simulink model "hw2_model"  (R2024b)
settings: Solver=FixedStepAuto  StartTime=0.0  StopTime=T  FixedStep=dt  RelTol=1e-3
undefined symbols (not defined in the file): dt, L, P0, Q, R, x0
settings Model: Creator=Atakan  LastModifiedBy=Atakan

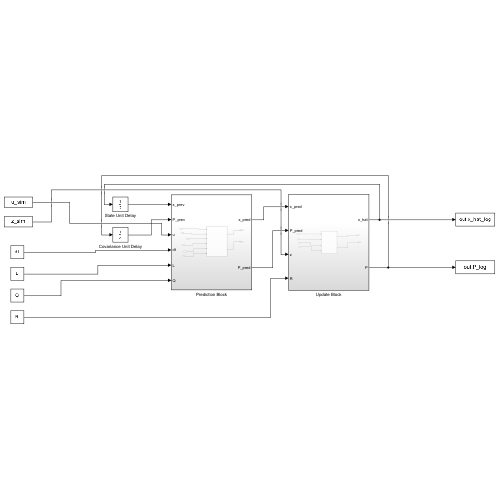
[thumbnail: Simulink's stored preview of the top-level diagram]
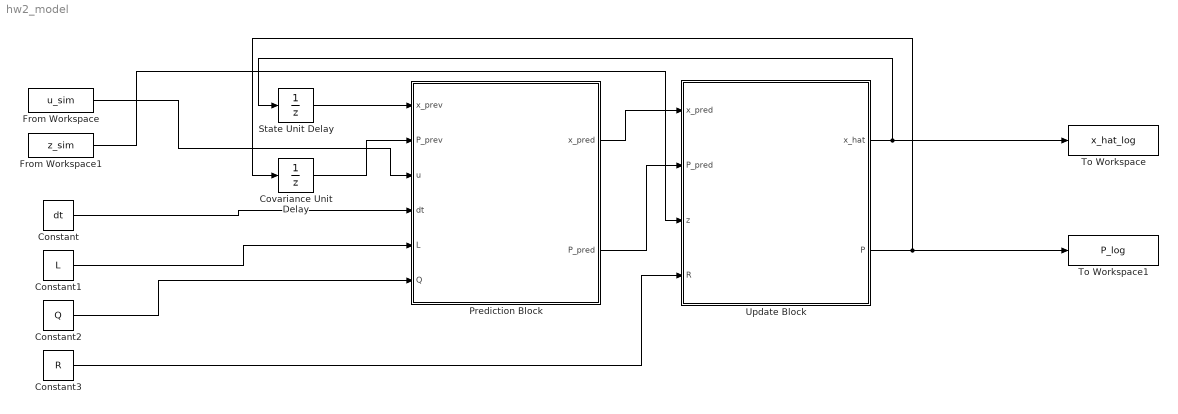
== system hw2_model ==
  Constant : Constant  Value=dt
  Constant1 : Constant  Value=L
  Constant2 : Constant  Value=Q
  Constant3 : Constant  Value=R
  Covariance Unit Delay : UnitDelay  InitialCondition=P0  SampleTime=dt  HasFrameUpgradeWarning=on
  From Workspace : FromWorkspace  VariableName=u_sim
  From Workspace1 : FromWorkspace  VariableName=z_sim
  Prediction Block : Subsystem
  State Unit Delay : UnitDelay  InitialCondition=x0  SampleTime=dt  HasFrameUpgradeWarning=on
  To Workspace : ToWorkspace  VariableName=x_hat_log  SampleTime=-1
  To Workspace1 : ToWorkspace  VariableName=P_log  SampleTime=-1
  Update Block : Subsystem
  wires:
  State Unit Delay/1 -> Prediction Block/1(x_prev)
  Covariance Unit Delay/1 -> Prediction Block/2(P_prev)
  From Workspace/1 -> Prediction Block/3(u)
  Constant/1 -> Prediction Block/4(dt)
  Constant1/1 -> Prediction Block/5(L)
  Constant2/1 -> Prediction Block/6(Q)
  Prediction Block/1(x_pred) -> Update Block/1(x_pred)
  Prediction Block/2(P_pred) -> Update Block/2(P_pred)
  From Workspace1/1 -> Update Block/3(z)
  Constant3/1 -> Update Block/4(R)
  Update Block/1(x_hat) -> State Unit Delay/1, To Workspace/1
  Update Block/2(P) -> To Workspace1/1, Covariance Unit Delay/1

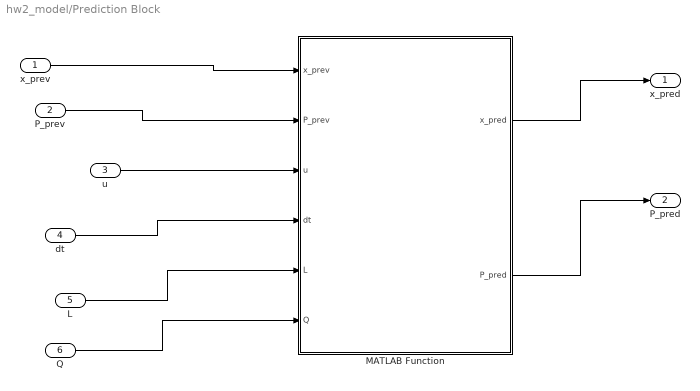
== system hw2_model/Prediction Block ==
  x_prev : Inport
  P_prev : Inport  Port=2
  u : Inport  Port=3
  dt : Inport  Port=4
  L : Inport  Port=5
  Q : Inport  Port=6
  MATLAB Function : MATLAB Function  TreatAsAtomicUnit=on
  x_pred : Outport
  P_pred : Outport  Port=2
  wires:
  x_prev/1 -> MATLAB Function/1(x_prev)
  P_prev/1 -> MATLAB Function/2(P_prev)
  u/1 -> MATLAB Function/3(u)
  dt/1 -> MATLAB Function/4(dt)
  L/1 -> MATLAB Function/5(L)
  Q/1 -> MATLAB Function/6(Q)
  MATLAB Function/1(x_pred) -> x_pred/1
  MATLAB Function/2(P_pred) -> P_pred/1

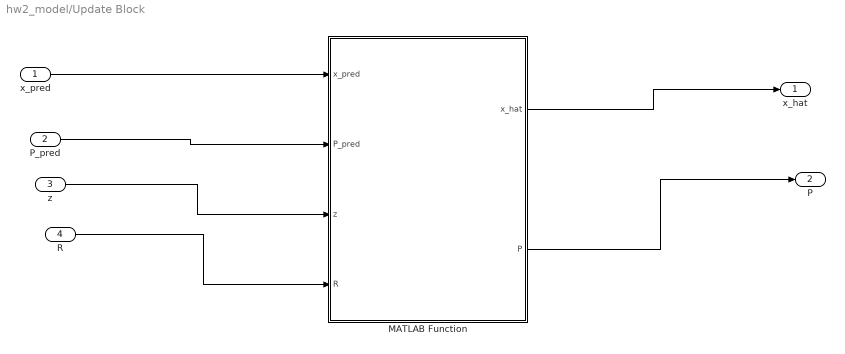
== system hw2_model/Update Block ==
  x_pred : Inport
  P_pred : Inport  Port=2
  z : Inport  Port=3
  R : Inport  Port=4
  MATLAB Function : MATLAB Function  TreatAsAtomicUnit=on
  x_hat : Outport
  P : Outport  Port=2
  wires:
  x_pred/1 -> MATLAB Function/1(x_pred)
  P_pred/1 -> MATLAB Function/2(P_pred)
  z/1 -> MATLAB Function/3(z)
  R/1 -> MATLAB Function/4(R)
  MATLAB Function/1(x_hat) -> x_hat/1
  MATLAB Function/2(P) -> P/1

== matlab function hw2_model/Update Block/MATLAB Function ==
  data: x_pred input; x_hat output; P_pred input; z input; R input; P output
function [x_hat, P] = update_block(x_pred, P_pred, z, R)
% EKF update step for GPS-like position measurement

% Make measurement vector safe
z = z(:);

% Measurement matrix
H = [1, 0, 0;
     0, 1, 0];

% Predicted measurement
z_pred = H*x_pred;

% Innovation
y = z - z_pred;

% Innovation covariance
S = H*P_pred*H' + R;

% Kalman gain
K = (P_pred*H') / S;

% State update
x_hat = x_pred + K*y;

% Normalize heading angle
x_hat(3) = atan2(sin(x_hat(3)), cos(x_hat(3)));

% Covariance update
I = eye(3);
P = (I - K*H)*P_pred;
end

== matlab function hw2_model/Prediction Block/MATLAB Function ==
  data: x_prev input; P_prev input; u input; x_pred output; dt input; L input; Q input; P_pred output
function [x_pred, P_pred] = prediction_block(x_prev, P_prev, u, dt, L, Q)
% EKF prediction step for kinematic bicycle model

% Make input vector safe
u = u(:);

% States
px    = x_prev(1);
py    = x_prev(2);
theta = x_prev(3);

% Inputs
delta = u(1);
v     = u(2);

% Nonlinear state prediction
x_pred = zeros(3,1);

x_pred(1) = px + v*cos(theta)*dt;
x_pred(2) = py + v*sin(theta)*dt;
x_pred(3) = theta + (v/L)*tan(delta)*dt;

% Normalize heading angle
x_pred(3) = atan2(sin(x_pred(3)), cos(x_pred(3)));

% Jacobian matrix
F = [1, 0, -v*sin(theta)*dt;
     0, 1,  v*cos(theta)*dt;
     0, 0,  1];

% Covariance prediction
P_pred = F*P_prev*F' + Q;
end
